simulink model "mas508_cw34_example3"  (R2021b)
settings: Solver=FixedStepAuto  StartTime=0.0  StopTime=6  FixedStep=1e-3  RelTol=1e-3
values from neighbouring files (symbols this model uses):
  b = 20    [mas508_cw34.m]    (also in mas508_lab2_exercise3_4.m = 0.06)
  k = 1000    [Lab6_example2_3.m]    (also in mas508_cw34.m = 1200; mas508_lab2_exercise2.m = 100; mas508_lab2_exercise3_4.m = 6)
  m = 11.2    [mas508_cw34.m]
libraries: simulink_extras x2
settings Model: Creator=rtavares  LastModifiedBy=faisala
settings SolverCC: AlgebraicLoopSolver=TrustRegion
settings DataIOCC: ReturnWorkspaceOutputs=off
settings DebuggingCC: SFMachineParentedDataDiag=warning

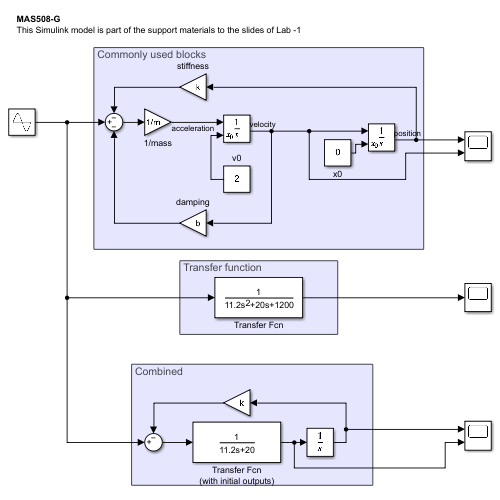
[thumbnail: Simulink's stored preview of the top-level diagram]
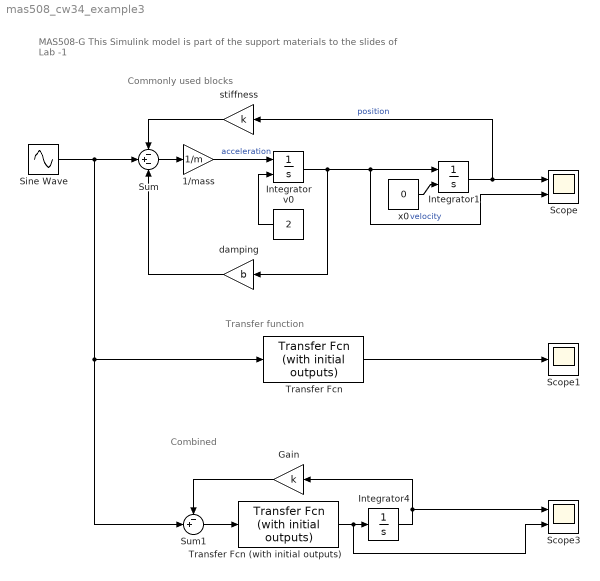
== system mas508_cw34_example3 ==
  note: Combined
  note: Transfer function
  note: Commonly used blocks
  note: MAS508-G
      | This Simulink model is part of the support materials to the slides of Lab -1
  1/mass : Gain  Gain=1/m
  Gain : Gain  Gain=k
  Integrator : Integrator  InitialConditionSource=external
  Integrator1 : Integrator  InitialConditionSource=external  InitialCondition=1.5
  Integrator4 : Integrator
  Scope : Scope  NumInputPorts=2
  Scope1 : Scope
  Scope3 : Scope  NumInputPorts=2
  Sine Wave : Sin  Amplitude=200  Frequency=2*pi*3  SampleTime=0
  Sum : Sum  Inputs=-+-
  Sum1 : Sum  Inputs=-+|
  Transfer Fcn : simulink_extras/Additional Linear/Transfer Fcn (with initial outputs)  N=[1]  D=[m b k]  Y0=0  U0=0
  Transfer Fcn (with initial outputs) : simulink_extras/Additional Linear/Transfer Fcn (with initial outputs)  N=[1]  D=[m b]  Y0=2  U0=0
  damping : Gain  Gain=b
  stiffness : Gain  Gain=k
  v0 : Constant  Value=2
  x0 : Constant  Value=0
  wires:
  stiffness/1 -> Sum/1
  Integrator1/1 -> stiffness/1, Scope/1  "position"
  Sum/1 -> 1/mass/1
  v0/1 -> Integrator/2
  damping/1 -> Sum/3
  1/mass/1 -> Integrator/1  "acceleration"
  x0/1 -> Integrator1/2
  Integrator/1 -> Integrator1/1, Scope/2, damping/1  "velocity"
  Transfer Fcn/1 -> Scope1/1
  Integrator4/1 -> Gain/1, Scope3/1
  Transfer Fcn (with initial outputs)/1 -> Scope3/2, Integrator4/1
  Sine Wave/1 -> Transfer Fcn/1, Sum1/2, Sum/2
  Sum1/1 -> Transfer Fcn (with initial outputs)/1
  Gain/1 -> Sum1/1
